simulink model "final"  (R2020a)
(part 8 of 10)

  "pd{1,1}"/1 -> dotprod1000/2, dotprod999/2, dotprod998/2, dotprod997/2, dotprod996/2, dotprod995/2, dotprod994/2, dotprod993/2, dotprod992/2, dotprod991/2, dotprod990/2, dotprod989/2, dotprod988/2, dotprod987/2, dotprod986/2, dotprod985/2, dotprod984/2, dotprod983/2, dotprod982/2, dotprod981/2, dotprod980/2, dotprod979/2, dotprod978/2, dotprod977/2, dotprod976/2, dotprod975/2, dotprod974/2, dotprod973/2, dotprod972/2, dotprod971/2, dotprod970/2, dotprod969/2, dotprod968/2, dotprod967/2, dotprod966/2, dotprod965/2, dotprod964/2, dotprod963/2, dotprod962/2, dotprod961/2, dotprod960/2, dotprod959/2, dotprod958/2, dotprod957/2, dotprod956/2, dotprod955/2, dotprod954/2, dotprod953/2, dotprod952/2, dotprod951/2, dotprod950/2, dotprod949/2, dotprod948/2, dotprod947/2, dotprod946/2, dotprod945/2, dotprod944/2, dotprod943/2, dotprod942/2, dotprod941/2, dotprod940/2, dotprod939/2, dotprod938/2, dotprod937/2, dotprod936/2, dotprod935/2, dotprod934/2, dotprod933/2, dotprod932/2, dotprod931/2, dotprod930/2, dotprod929/2, dotprod928/2, dotprod927/2, dotprod926/2, dotprod925/2, dotprod924/2, dotprod923/2, dotprod922/2, dotprod921/2, dotprod920/2, dotprod919/2, dotprod918/2, dotprod917/2, dotprod916/2, dotprod915/2, dotprod914/2, dotprod913/2, dotprod912/2, dotprod911/2, dotprod910/2, dotprod909/2, dotprod908/2, dotprod907/2, dotprod906/2, dotprod905/2, dotprod904/2, dotprod903/2, dotprod902/2, dotprod901/2, dotprod900/2, dotprod899/2, dotprod898/2, dotprod897/2, dotprod896/2, dotprod895/2, dotprod894/2, dotprod893/2, dotprod892/2, dotprod891/2, dotprod890/2, dotprod889/2, dotprod888/2, dotprod887/2, dotprod886/2, dotprod885/2, dotprod884/2, dotprod883/2, dotprod882/2, dotprod881/2, dotprod880/2, dotprod879/2, dotprod878/2, dotprod877/2, dotprod876/2, dotprod875/2, dotprod874/2, dotprod873/2, dotprod872/2, dotprod871/2, dotprod870/2, dotprod869/2, dotprod868/2, dotprod867/2, dotprod866/2, dotprod865/2, dotprod864/2, dotprod863/2, dotprod862/2, dotprod861/2, dotprod860/2, dotprod859/2, dotprod858/2, dotprod857/2, dotprod856/2, dotprod855/2, dotprod854/2, dotprod853/2, dotprod852/2, dotprod851/2, dotprod850/2, dotprod849/2, dotprod848/2, dotprod847/2, dotprod846/2, dotprod845/2, dotprod844/2, dotprod843/2, dotprod842/2, dotprod841/2, dotprod840/2, dotprod839/2, dotprod838/2, dotprod837/2, dotprod836/2, dotprod835/2, dotprod834/2, dotprod833/2, dotprod832/2, dotprod831/2, dotprod830/2, dotprod829/2, dotprod828/2, dotprod827/2, dotprod826/2, dotprod825/2, dotprod824/2, dotprod823/2, dotprod822/2, dotprod821/2, dotprod820/2, dotprod819/2, dotprod818/2, dotprod817/2, dotprod816/2, dotprod815/2, dotprod814/2, dotprod813/2, dotprod812/2, dotprod811/2, dotprod810/2, dotprod809/2, dotprod808/2, dotprod807/2, dotprod806/2, dotprod805/2, dotprod804/2, dotprod803/2, dotprod802/2, dotprod801/2, dotprod800/2, dotprod799/2, dotprod798/2, dotprod797/2, dotprod796/2, dotprod795/2, dotprod794/2, dotprod793/2, dotprod792/2, dotprod791/2, dotprod790/2, dotprod789/2, dotprod788/2, dotprod787/2, dotprod786/2, dotprod785/2, dotprod784/2, dotprod783/2, dotprod782/2, dotprod781/2, dotprod780/2, dotprod779/2, dotprod778/2, dotprod777/2, dotprod776/2, dotprod775/2, dotprod774/2, dotprod773/2, dotprod772/2, dotprod771/2, dotprod770/2, dotprod769/2, dotprod768/2, dotprod767/2, dotprod766/2, dotprod765/2, dotprod764/2, dotprod763/2, dotprod762/2, dotprod761/2, dotprod760/2, dotprod759/2, dotprod758/2, dotprod757/2, dotprod756/2, dotprod755/2, dotprod754/2, dotprod753/2, dotprod752/2, dotprod751/2, dotprod750/2, dotprod749/2, dotprod748/2, dotprod747/2, dotprod746/2, dotprod745/2, dotprod744/2, dotprod743/2, dotprod742/2, dotprod741/2, dotprod740/2, dotprod739/2, dotprod738/2, dotprod737/2, dotprod736/2, dotprod735/2, dotprod734/2, dotprod733/2, dotprod732/2, dotprod731/2, dotprod730/2, dotprod729/2, dotprod728/2, dotprod727/2, dotprod726/2, dotprod725/2, dotprod724/2, dotprod723/2, dotprod722/2, dotprod721/2, dotprod720/2, dotprod719/2, dotprod718/2, dotprod717/2, dotprod716/2, dotprod715/2, dotprod714/2, dotprod713/2, dotprod712/2, dotprod711/2, dotprod710/2, dotprod709/2, dotprod708/2, dotprod707/2, dotprod706/2, dotprod705/2, dotprod704/2, dotprod703/2, dotprod702/2, dotprod701/2, dotprod700/2, dotprod699/2, dotprod698/2, dotprod697/2, dotprod696/2, dotprod695/2, dotprod694/2, dotprod693/2, dotprod692/2, dotprod691/2, dotprod690/2, dotprod689/2, dotprod688/2, dotprod687/2, dotprod686/2, dotprod685/2, dotprod684/2, dotprod683/2, dotprod682/2, dotprod681/2, dotprod680/2, dotprod679/2, dotprod678/2, dotprod677/2, dotprod676/2, dotprod675/2, dotprod674/2, dotprod673/2, dotprod672/2, dotprod671/2, dotprod670/2, dotprod669/2, dotprod668/2, dotprod667/2, dotprod666/2, dotprod665/2, dotprod664/2, dotprod663/2, dotprod662/2, dotprod661/2, dotprod660/2, dotprod659/2, dotprod658/2, dotprod657/2, dotprod656/2, dotprod655/2, dotprod654/2, dotprod653/2, dotprod652/2, dotprod651/2, dotprod650/2, dotprod649/2, dotprod648/2, dotprod647/2, dotprod646/2, dotprod645/2, dotprod644/2, dotprod643/2, dotprod642/2, dotprod641/2, dotprod640/2, dotprod639/2, dotprod638/2, dotprod637/2, dotprod636/2, dotprod635/2, dotprod634/2, dotprod633/2, dotprod632/2, dotprod631/2, dotprod630/2, dotprod629/2, dotprod628/2, dotprod627/2, dotprod626/2, dotprod625/2, dotprod624/2, dotprod623/2, dotprod622/2, dotprod621/2, dotprod620/2, dotprod619/2, dotprod618/2, dotprod617/2, dotprod616/2, dotprod615/2, dotprod614/2, dotprod613/2, dotprod612/2, dotprod611/2, dotprod610/2, dotprod609/2, dotprod608/2, dotprod607/2, dotprod606/2, dotprod605/2, dotprod604/2, dotprod603/2, dotprod602/2, dotprod601/2, dotprod600/2, dotprod599/2, dotprod598/2, dotprod597/2, dotprod596/2, dotprod595/2, dotprod594/2, dotprod593/2, dotprod592/2, dotprod591/2, dotprod590/2, dotprod589/2, dotprod588/2, dotprod587/2, dotprod586/2, dotprod585/2, dotprod584/2, dotprod583/2, dotprod582/2, dotprod581/2, dotprod580/2, dotprod579/2, dotprod578/2, dotprod577/2, dotprod576/2, dotprod575/2, dotprod574/2, dotprod573/2, dotprod572/2, dotprod571/2, dotprod570/2, dotprod569/2, dotprod568/2, dotprod567/2, dotprod566/2, dotprod565/2, dotprod564/2, dotprod563/2, dotprod562/2, dotprod561/2, dotprod560/2, dotprod559/2, dotprod558/2, dotprod557/2, dotprod556/2, dotprod555/2, dotprod554/2, dotprod553/2, dotprod552/2, dotprod551/2, dotprod550/2, dotprod549/2, dotprod548/2, dotprod547/2, dotprod546/2, dotprod545/2, dotprod544/2, dotprod543/2, dotprod542/2, dotprod541/2, dotprod540/2, dotprod539/2, dotprod538/2, dotprod537/2, dotprod536/2, dotprod535/2, dotprod534/2, dotprod533/2, dotprod532/2, dotprod531/2, dotprod530/2, dotprod529/2, dotprod528/2, dotprod527/2, dotprod526/2, dotprod525/2, dotprod524/2, dotprod523/2, dotprod522/2, dotprod521/2, dotprod520/2, dotprod519/2, dotprod518/2, dotprod517/2, dotprod516/2, dotprod515/2, dotprod514/2, dotprod513/2, dotprod512/2, dotprod511/2, dotprod510/2, dotprod509/2, dotprod508/2, dotprod507/2, dotprod506/2, dotprod505/2, dotprod504/2, dotprod503/2, dotprod502/2, dotprod501/2, dotprod500/2, dotprod499/2, dotprod498/2, dotprod497/2, dotprod496/2, dotprod495/2, dotprod494/2, dotprod493/2, dotprod492/2, dotprod491/2, dotprod490/2, dotprod489/2, dotprod488/2, dotprod487/2, dotprod486/2, dotprod485/2, dotprod484/2, dotprod483/2, dotprod482/2, dotprod481/2, dotprod480/2, dotprod479/2, dotprod478/2, dotprod477/2, dotprod476/2, dotprod475/2, dotprod474/2, dotprod473/2, dotprod472/2, dotprod471/2, dotprod470/2, dotprod469/2, dotprod468/2, dotprod467/2, dotprod466/2, dotprod465/2, dotprod464/2, dotprod463/2, dotprod462/2, dotprod461/2, dotprod460/2, dotprod459/2, dotprod458/2, dotprod457/2, dotprod456/2, dotprod455/2, dotprod454/2, dotprod453/2, dotprod452/2, dotprod451/2, dotprod450/2, dotprod449/2, dotprod448/2, dotprod447/2, dotprod446/2, dotprod445/2, dotprod444/2, dotprod443/2, dotprod442/2, dotprod441/2, dotprod440/2, dotprod439/2, dotprod438/2, dotprod437/2, dotprod436/2, dotprod435/2, dotprod434/2, dotprod433/2, dotprod432/2, dotprod431/2, dotprod430/2, dotprod429/2, dotprod428/2, dotprod427/2, dotprod426/2, dotprod425/2, dotprod424/2, dotprod423/2, dotprod422/2, dotprod421/2, dotprod420/2, dotprod419/2, dotprod418/2, dotprod417/2, dotprod416/2, dotprod415/2, dotprod414/2, dotprod413/2, dotprod412/2, dotprod411/2, dotprod410/2, dotprod409/2, dotprod408/2, dotprod407/2, dotprod406/2, dotprod405/2, dotprod404/2, dotprod403/2, dotprod402/2, dotprod401/2, dotprod400/2, dotprod399/2, dotprod398/2, dotprod397/2, dotprod396/2, dotprod395/2, dotprod394/2, dotprod393/2, dotprod392/2, dotprod391/2, dotprod390/2, dotprod389/2, dotprod388/2, dotprod387/2, dotprod386/2, dotprod385/2, dotprod384/2, dotprod383/2, dotprod382/2, dotprod381/2, dotprod380/2, dotprod379/2, dotprod378/2, dotprod377/2, dotprod376/2, dotprod375/2, dotprod374/2, dotprod373/2, dotprod372/2, dotprod371/2, dotprod370/2, dotprod369/2, dotprod368/2, dotprod367/2, dotprod366/2, dotprod365/2, dotprod364/2, dotprod363/2, dotprod362/2, dotprod361/2, dotprod360/2, dotprod359/2, dotprod358/2, dotprod357/2, dotprod356/2, dotprod355/2, dotprod354/2, dotprod353/2, dotprod352/2, dotprod351/2, dotprod350/2, dotprod349/2, dotprod348/2, dotprod347/2, dotprod346/2, dotprod345/2, dotprod344/2, dotprod343/2, dotprod342/2, dotprod341/2, dotprod340/2, dotprod339/2, dotprod338/2, dotprod337/2, dotprod336/2, dotprod335/2, dotprod334/2, dotprod333/2, dotprod332/2, dotprod331/2, dotprod330/2, dotprod329/2, dotprod328/2, dotprod327/2, dotprod326/2, dotprod325/2, dotprod324/2, dotprod323/2, dotprod322/2, dotprod321/2, dotprod320/2, dotprod319/2, dotprod318/2, dotprod317/2, dotprod316/2, dotprod315/2, dotprod314/2, dotprod313/2, dotprod312/2, dotprod311/2, dotprod310/2, dotprod309/2, dotprod308/2, dotprod307/2, dotprod306/2, dotprod305/2, dotprod304/2, dotprod303/2, dotprod302/2, dotprod301/2, dotprod300/2, dotprod299/2, dotprod298/2, dotprod297/2, dotprod296/2, dotprod295/2, dotprod294/2, dotprod293/2, dotprod292/2, dotprod291/2, dotprod290/2, dotprod289/2, dotprod288/2, dotprod287/2, dotprod286/2, dotprod285/2, dotprod284/2, dotprod283/2, dotprod282/2, dotprod281/2, dotprod280/2, dotprod279/2, dotprod278/2, dotprod277/2, dotprod276/2, dotprod275/2, dotprod274/2, dotprod273/2, dotprod272/2, dotprod271/2, dotprod270/2, dotprod269/2, dotprod268/2, dotprod267/2, dotprod266/2, dotprod265/2, dotprod264/2, dotprod263/2, dotprod262/2, dotprod261/2, dotprod260/2, dotprod259/2, dotprod258/2, dotprod257/2, dotprod256/2, dotprod255/2, dotprod254/2, dotprod253/2, dotprod252/2, dotprod251/2, dotprod250/2, dotprod249/2, dotprod248/2, dotprod247/2, dotprod246/2, dotprod245/2, dotprod244/2, dotprod243/2, dotprod242/2, dotprod241/2, dotprod240/2, dotprod239/2, dotprod238/2, dotprod237/2, dotprod236/2, dotprod235/2, dotprod234/2, dotprod233/2, dotprod232/2, dotprod231/2, dotprod230/2, dotprod229/2, dotprod228/2, dotprod227/2, dotprod226/2, dotprod225/2, dotprod224/2, dotprod223/2, dotprod222/2, dotprod221/2, dotprod220/2, dotprod219/2, dotprod218/2, dotprod217/2, dotprod216/2, dotprod215/2, dotprod214/2, dotprod213/2, dotprod212/2, dotprod211/2, dotprod210/2, dotprod209/2, dotprod208/2, dotprod207/2, dotprod206/2, dotprod205/2, dotprod204/2, dotprod203/2, dotprod202/2, dotprod201/2, dotprod200/2, dotprod199/2, dotprod198/2, dotprod197/2, dotprod196/2, dotprod195/2, dotprod194/2, dotprod193/2, dotprod192/2, dotprod191/2, dotprod190/2, dotprod189/2, dotprod188/2, dotprod187/2, dotprod186/2, dotprod185/2, dotprod184/2, dotprod183/2, dotprod182/2, dotprod181/2, dotprod180/2, dotprod179/2, dotprod178/2, dotprod177/2, dotprod176/2, dotprod175/2, dotprod174/2, dotprod173/2, dotprod172/2, dotprod171/2, dotprod170/2, dotprod169/2, dotprod168/2, dotprod167/2, dotprod166/2, dotprod165/2, dotprod164/2, dotprod163/2, dotprod162/2, dotprod161/2, dotprod160/2, dotprod159/2, dotprod158/2, dotprod157/2, dotprod156/2, dotprod155/2, dotprod154/2, dotprod153/2, dotprod152/2, dotprod151/2, dotprod150/2, dotprod149/2, dotprod148/2, dotprod147/2, dotprod146/2, dotprod145/2, dotprod144/2, dotprod143/2, dotprod142/2, dotprod141/2, dotprod140/2, dotprod139/2, dotprod138/2, dotprod137/2, dotprod136/2, dotprod135/2, dotprod134/2, dotprod133/2, dotprod132/2, dotprod131/2, dotprod130/2, dotprod129/2, dotprod128/2, dotprod127/2, dotprod126/2, dotprod125/2, dotprod124/2, dotprod123/2, dotprod122/2, dotprod121/2, dotprod120/2, dotprod119/2, dotprod118/2, dotprod117/2, dotprod116/2, dotprod115/2, dotprod114/2, dotprod113/2, dotprod112/2, dotprod111/2, dotprod110/2, dotprod109/2, dotprod108/2, dotprod107/2, dotprod106/2, dotprod105/2, dotprod104/2, dotprod103/2, dotprod102/2, dotprod101/2, dotprod100/2, dotprod99/2, dotprod98/2, dotprod97/2, dotprod96/2, dotprod95/2, dotprod94/2, dotprod93/2, dotprod92/2, dotprod91/2, dotprod90/2, dotprod89/2, dotprod88/2, dotprod87/2, dotprod86/2, dotprod85/2, dotprod84/2, dotprod83/2, dotprod82/2, dotprod81/2, dotprod80/2, dotprod79/2, dotprod78/2, dotprod77/2, dotprod76/2, dotprod75/2, dotprod74/2, dotprod73/2, dotprod72/2, dotprod71/2, dotprod70/2, dotprod69/2, dotprod68/2, dotprod67/2, dotprod66/2, dotprod65/2, dotprod64/2, dotprod63/2, dotprod62/2, dotprod61/2, dotprod60/2, dotprod59/2, dotprod58/2, dotprod57/2, dotprod56/2, dotprod55/2, dotprod54/2, dotprod53/2, dotprod52/2, dotprod51/2, dotprod50/2, dotprod49/2, dotprod48/2, dotprod47/2, dotprod46/2, dotprod45/2, dotprod44/2, dotprod43/2, dotprod42/2, dotprod41/2, dotprod40/2, dotprod39/2, dotprod38/2, dotprod37/2, dotprod36/2, dotprod35/2, dotprod34/2, dotprod33/2, dotprod32/2, dotprod31/2, dotprod30/2, dotprod29/2, dotprod28/2, dotprod27/2, dotprod26/2, dotprod25/2, dotprod24/2, dotprod23/2, dotprod22/2, dotprod21/2, dotprod20/2, dotprod19/2, dotprod18/2, dotprod17/2, dotprod16/2, dotprod15/2, dotprod14/2, dotprod13/2, dotprod12/2, dotprod11/2, dotprod10/2, dotprod9/2, dotprod8/2, dotprod7/2, dotprod6/2, dotprod5/2, dotprod4/2, dotprod3/2, dotprod2/2, dotprod1/2
  "IW{1,1}(1,:)'"/1 -> dotprod1/1
